simulink model "BPSK_and_OFDM"  (R2024a)
settings: Solver=VariableStepAuto  StartTime=0.0  StopTime=10.0  RelTol=1e-3
libraries: commdigbbndpm3 x2, commofdm x2, commchan3 x1, commrandsrc3 x1, matrix_library x1
settings Model: Creator=Anusnekhaa Narendran  LastModifiedBy=Anusnekhaa Narendran

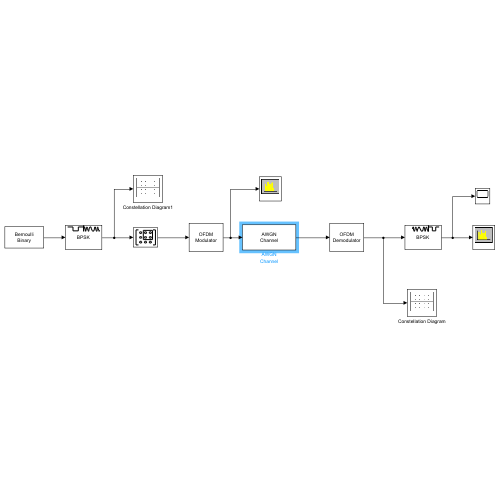
[thumbnail: Simulink's stored preview of the top-level diagram]
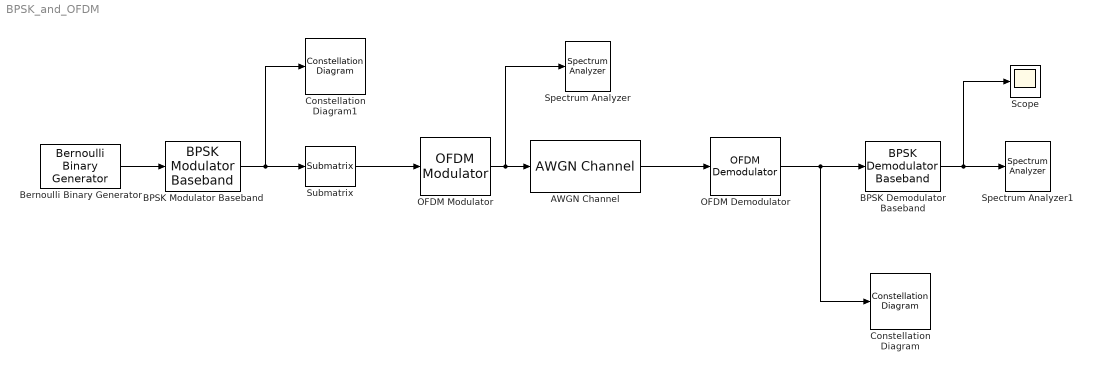
== system BPSK_and_OFDM ==
  AWGN Channel : commchan3/AWGN Channel  LegacyMode=off  NoiseMethod="Signal to noise ratio  (SNR)"  noiseMode="Signal to noise ratio  (SNR)"  EbNo=10  EsNo=10  SNR=10  BitsPerSymbol=1  SignalPower=1  SamplesPerSymbol=1  SymbolPeriod=1  VarianceSource=Parameter  Variance=1  RandomStream=Global stream  Seed=67  SimulateUsing=Code generation
  BPSK Demodulator Baseband : commdigbbndpm3/BPSK Demodulator Baseband  DecType=Hard decision  VarSource=Dialog  Variance=1  Ph=0  outDtype=boolean  derotateFactorWordLen=16  derotateFactorDataTypeStr=Inherit: Same word length as input  derotateFactorLastDataTypeStr=Inherit: Same word length as input
  BPSK Modulator Baseband : commdigbbndpm3/BPSK Modulator Baseband  Ph=0  outDtype=double  outWordLen=16  outUDDataType=sfix(16)  outFracLenMode=Best precision  outFracLen=15  outDataTypeStr=double  outLastDataTypeStr=double
  Bernoulli Binary Generator : commrandsrc3/Bernoulli Binary Generator  ProbabilityOfZero=0.5  SeedSource=Auto  Seed=0  SampleTime=1e-6  SamplesPerFrame=1000  OutputDataType=boolean  SimulateUsing=Interpreted execution
  Constellation Diagram : ConstellationDiagram  WindowPosition=[382.000000,84.000000,600.000000,600.000000,]  Visible=on  ScopeFrameLocation=window  XLimits=[-2.65,2.65]  YLimits=[-2.5,2.5]
  Constellation Diagram1 : ConstellationDiagram  WindowPosition=[382.000000,84.000000,600.000000,600.000000,]  Visible=on  ScopeFrameLocation=window
  OFDM Demodulator : commofdm/OFDM Demodulator  StatePerturbationForJacobian=1.0e-05  FFTLength=64  NumGuardBandCarriers=[6; 5]  RemoveDCCarrier=off  PilotOutputPort=off  PilotCarrierIndices=[12; 26; 40; 54]  CyclicPrefixLength=16  OversamplingFactor=1  NumSymbols=1  NumReceiveAntennas=1  SimulateUsing=Interpreted execution
  OFDM Modulator : commofdm/OFDM Modulator  StatePerturbationForJacobian=1.0e-05  FFTLength=64  NumGuardBandCarriers=[6; 5]  InsertDCNull=off  PilotInputPort=off  PilotCarrierIndices=[12; 26; 40; 54]  CyclicPrefixLength=16  Windowing=off  WindowLength=1  OversamplingFactor=1  NumSymbols=1  NumTransmitAntennas=1  SimulateUsing=Interpreted execution
  Scope : Scope
  Spectrum Analyzer : SpectrumAnalyzer  WindowPosition=[368.000000,182.000000,800.000000,500.000000,]  Visible=on  ScopeFrameLocation=window  YLimits=[-43.48035015,-11.32204683]
  Spectrum Analyzer1 : SpectrumAnalyzer  WindowPosition=[368.000000,182.000000,800.000000,500.000000,]  Visible=on  ScopeFrameLocation=window  YLimits=[-13.97439658,28.21685387]
  Submatrix : matrix_library/Submatrix  RowSpan=Range of rows  RowStartMode=Index  RowStartIndex=1  RowEndMode=Index  RowEndIndex=53  ColSpan=Range of columns  ColStartMode=Index  ColStartIndex=1  ColEndMode=Index  ColEndIndex=1
  wires:
  Bernoulli Binary Generator/1 -> BPSK Modulator Baseband/1
  BPSK Modulator Baseband/1 -> Constellation Diagram1/1, Submatrix/1
  Submatrix/1 -> OFDM Modulator/1
  OFDM Modulator/1 -> Spectrum Analyzer/1, AWGN Channel/1
  AWGN Channel/1 -> OFDM Demodulator/1
  BPSK Demodulator Baseband/1 -> Scope/1, Spectrum Analyzer1/1
  OFDM Demodulator/1 -> Constellation Diagram/1, BPSK Demodulator Baseband/1
